simulink model "grid_afe_n"  (R2026a)
settings: Solver=ode23tb  StopTime=simlength  FixedStep=tc  MaxStep=glb_time.tc
values from neighbouring files (symbols this model uses):
  afe_ctrl = ctrl_afe_setup(glb_time.ts_afe, grid_emu.omega_grid_nom)    [init_model.m]
  afe_pwm_phase_shift_mod1 = 0    [init_model.m]
  afe_pwm_phase_shift_mod2 = 0    [init_model.m]
  afe_pwm_phase_shift_mod3 = 0    [init_model.m]
  afe_pwm_phase_shift_mod4 = 0    [init_model.m]
  filters = setup_global_filters(glb_time.ts_afe, glb_time.ts_inv, glb_time.ts_dab, glb_time.tc)    [init_model.m]
  frt_data = frt_settings(test_index, test_subindex, asymmetric_error_type,      enable_frt_1, enable_frt_2, start_time_LVRT, deepPOSxi, deepPOSeta, deepNEGxi, deepNEGeta)    [init_model.m]
  glb_time = timing_setup(fpwm_afe, trgo_afe, fpwm_inv, trgo_inv, fpwm_single_phase_inv, trgo_single_phase_inv, fpwm_dab, trgo_dab,      fpwm_psfbc, trgo_psfbc, fpwm_isop_rail, trgo_isop_rail, fpwm_cllc, trgo_cllc, t_measure, tc_factor, tc_decimation, delay_pwm, dead_time_afe,      dead_time_inv, dead_time_single_phase_inv, dead_time_dab, dead_time_psfbc, dead_time_isop_rail, dead_time_cllc)    [init_model.m]
  grid_emu = grid_three_phase_emulator('Dyn11', delta_star, grid_nominal_power, application_voltage, us1, us2, fgrid,                  eq_grid_inductance, eq_grid_resistance, eta, ucc, i1m, p_iron, n1, n2, core_area, core_length, mur,                  up_xi_pu_ref, up_eta_pu_ref, un_xi_pu_ref, un_eta_pu_ref)    [init_model.m]
  i_react_pos_ref_2 = -ixi_ref_mod1*tan(acos(0.95))    [init_model.m]
  i_react_pos_ref_3 = ixi_ref_mod1*tan(acos(0.95))    [init_model.m]
  ixi_ref_mod1 = -0.85    [init_model.m]
  ixi_ref_mod2 = -0.85    [init_model.m]
  ixi_ref_mod3 = -0.85    [init_model.m]
  ixi_ref_mod4 = -0.85    [init_model.m]
  ki_align = 18    [init_model.m]
  kp_align = 0.25    [init_model.m]
  lim_down_align = -0.05    [init_model.m]
  lim_up_align = 0.05    [init_model.m]
  mavarage_filter_frequency_base_order = 2    [init_model.m]
  time_gain_afe_module_1 = 1.0002    [init_model.m]
  time_gain_afe_module_2 = 1.0015    [init_model.m]
  time_gain_afe_module_3 = 0.9988    [init_model.m]
  time_gain_afe_module_4 = 1.0020    (= 1.002)    [init_model.m]
  time_i_react_pos_ref_1 = start_time_LVRT + error_length + 0.335    [init_model.m]
  time_i_react_pos_ref_2 = time_i_react_pos_ref_1 + 0.5    (= 0.5)    [init_model.m]
  u_cm_comp_mod1 = 0    [init_model.m]
  u_cm_comp_mod2 = -1    [init_model.m]
  u_cm_comp_mod3 = -1    [init_model.m]
  u_cm_comp_mod4 = -1    [init_model.m]
undefined symbols (not defined in the file or in its folder): hwdata, magnitude
libraries: fl_lib x113, nesl_utility x75, moving_average_filter x40, moving_average_filter_cc x32, sl_discontinuities x12, linear_double_integrator_observer_ccaller x8, discrete_time_low_pass_filter x4, threephase_inductor_lib x4, dclink_for_two_levels x4, three_phase_pwm_modulator x4, three_phase_inverter_ideal_switch_based_model x4, three_phase_inverter_igbt_advanced_thermal_model x4
(part 16 of 19)

== system grid_afe_n/afe_abc_mod4/AFE_control/afe_control/grid_voltage_phase_lock_loops/FHT-PLL/pll_stageA/filter_and_transformation ==
  ug_a : Inport
  ug_b : Inport  Port=2
  ug_c : Inport  Port=3
  Bus Creator : BusCreator  Inputs=2
  Bus Creator1 : BusCreator  Inputs=3
  Bus Creator2 : BusCreator  Inputs=2
  Bus Creator3 : BusCreator  Inputs=3
  Bus Creator4 : BusCreator  Inputs=3
  FHTalpha : Subsystem
  FHTbeta : Subsystem
  FHTdqPLL : Scope  NumInputPorts=2
      settings: ActiveDisplayYMinimum=-1.5258214459194912  ActiveDisplayYMaximum=1.5258228058860459  DataLoggingVariableName=ScopeData12
  Gain : Gain  Gain=-1/2
  Gain1 : Gain  Gain=-1/2
  Sum : Sum  Inputs=|++
  Sum1 : Sum  Inputs=-+|
  To Workspace1 : ToWorkspace  VariableName=ugd_alpha_sim  SampleTime=-1
      settings: MaxDataPoints=glb_time.Ns_afe
  To Workspace2 : ToWorkspace  VariableName=ugd_beta_sim  SampleTime=-1
      settings: MaxDataPoints=glb_time.Ns_afe
  To Workspace3 : ToWorkspace  VariableName=u_fht_alpha_sim  SampleTime=-1
      settings: MaxDataPoints=glb_time.Ns_afe
  To Workspace4 : ToWorkspace  VariableName=v_fht_alpha_sim  SampleTime=-1
      settings: MaxDataPoints=glb_time.Ns_afe
  To Workspace5 : ToWorkspace  VariableName=u_fhtsr_alpha_sim  SampleTime=-1
      settings: MaxDataPoints=glb_time.Ns_afe
  To Workspace6 : ToWorkspace  VariableName=u_fhtsr_beta_sim  SampleTime=-1
      settings: MaxDataPoints=glb_time.Ns_afe
  To Workspace7 : ToWorkspace  VariableName=u_fht_beta_sim  SampleTime=-1
      settings: MaxDataPoints=glb_time.Ns_afe
  To Workspace8 : ToWorkspace  VariableName=v_fht_beta_sim  SampleTime=-1
      settings: MaxDataPoints=glb_time.Ns_afe
  To Workspace9 : ToWorkspace  VariableName=ugd_abc_grid_sim  SampleTime=-1
      settings: MaxDataPoints=glb_time.Ns_afe
  abc2alphabeta : MATLAB Function  TreatAsAtomicUnit=on
  grid_voltages : Scope  NumInputPorts=3
      settings: ActiveDisplayYMinimum=-1.3618303835391998  ActiveDisplayYMaximum=1.3331545889377594  DataLoggingVariableName=ScopeData13
  ug_alpha : Outport  VectorParamsAs1DForOutWhenUnconnected=off
  ug_beta : Outport  Port=2  VectorParamsAs1DForOutWhenUnconnected=off
  wires:
  Bus Creator3/1 -> To Workspace9/1
  Bus Creator2/1 -> Bus Creator1/2  "FHTbeta"
  Bus Creator/1 -> Bus Creator4/2  "FHTalpha"
  Bus Creator4/1 -> FHTdqPLL/1
  Bus Creator1/1 -> FHTdqPLL/2
  FHTalpha/2(uq_hat) -> Bus Creator/2, To Workspace4/1, Sum1/1  "v_fht_alpha"
  FHTbeta/2(uq_hat) -> Bus Creator2/2, To Workspace8/1, Sum/2  "v_fht_beta"
  Gain/1 -> ug_alpha/1, To Workspace5/1, Bus Creator4/3  "u_fhtsr_alpha"
  Gain1/1 -> ug_beta/1, To Workspace6/1, Bus Creator1/3  "u_fhtsr_beta"
  Sum1/1 -> Gain1/1
  FHTbeta/1(ud_hat) -> Bus Creator2/1, To Workspace7/1, Sum1/2  "u_fht_beta"
  Sum/1 -> Gain/1
  FHTalpha/1(ud_hat) -> Sum/1, Bus Creator/1, To Workspace3/1  "u_fht_alpha"
  abc2alphabeta/2(beta) -> Bus Creator1/1, To Workspace2/1, FHTbeta/1(u)  "u_grid_beta"
  abc2alphabeta/1(alpha) -> Bus Creator4/1, FHTalpha/1(u), To Workspace1/1  "u_grid_alpha"
  ug_a/1 -> abc2alphabeta/1(a), grid_voltages/1, Bus Creator3/1  "ugd_a"
  ug_c/1 -> abc2alphabeta/3(c), grid_voltages/3, Bus Creator3/3  "ugd_c"
  ug_b/1 -> abc2alphabeta/2(b), grid_voltages/2, Bus Creator3/2  "ugd_b"

== system grid_afe_n/afe_abc_mod4/AFE_control/afe_control/grid_voltage_phase_lock_loops/FHT-PLL/pll_stageA/sequences ==
  u_grid_alpha : Inport
  u_grid_beta : Inport  Port=2
  phase_angle : Inport  Port=3
  alphabeta2xieta : MATLAB Function  TreatAsAtomicUnit=on
  u_grid_xi : Outport
  u_grid_eta : Outport  Port=2
  wires:
  phase_angle/1 -> alphabeta2xieta/3(gamma)  "phase_angle"
  u_grid_beta/1 -> alphabeta2xieta/2(beta)  "u_grid_beta"
  u_grid_alpha/1 -> alphabeta2xieta/1(alpha)  "u_grid_alpha"
  alphabeta2xieta/2(eta) -> u_grid_eta/1  "u_grid_eta"
  alphabeta2xieta/1(xi) -> u_grid_xi/1  "u_grid_xi"

== system grid_afe_n/afe_abc_mod4/AFE_control/afe_control/grid_voltage_phase_lock_loops/FHT-PLL/pll_stageB/double_integrator_observer ==
  theta : Inport
  Gain : Gain  Gain=afe_ctrl.di_obs.Ldso  Multiplication=Matrix(K*u)
  Gain1 : Gain  Gain=afe_ctrl.di_obs.Adso  Multiplication=Matrix(K*u)
  Gain2 : Gain  Gain=afe_ctrl.di_obs.Cso  Multiplication=Matrix(K*u)
  Selector : Selector  InputPortWidth=2  IndexOptions=Index vector (dialog)  Indices=2  OutputSizes=1
  Sum : Sum  Inputs=-+|
  Sum1 : Sum  Inputs=|++
  Unit Delay : UnitDelay  SampleTime=-1
  bounder1 : MATLAB Function  TreatAsAtomicUnit=on
  bounder2 : MATLAB Function  TreatAsAtomicUnit=on
  omega_hat : Outport
  wires:
  bounder2/1(y) -> Sum/1  "theta_hat_bounded"
  bounder1/1(y) -> Gain/1
  theta/1 -> Sum/2  "theta"
  Unit Delay/1 -> Gain2/1, Selector/1, Gain1/1
  Sum/1 -> bounder1/1(u)  "e"
  Sum1/1 -> Unit Delay/1
  Gain1/1 -> Sum1/2
  Gain2/1 -> bounder2/1(u)  "theta_hat"
  Selector/1 -> omega_hat/1
  Gain/1 -> Sum1/1

== system grid_afe_n/afe_abc_mod4/AFE_control/afe_control/grid_voltage_phase_lock_loops/FHT-PLL_simulink/pll_stageA/filter_and_transformation ==
  ug_a : Inport
  ug_b : Inport  Port=2
  ug_c : Inport  Port=3
  Bus Creator : BusCreator  Inputs=2
  Bus Creator1 : BusCreator  Inputs=3
  Bus Creator2 : BusCreator  Inputs=2
  Bus Creator4 : BusCreator  Inputs=3
  FHTalpha : Subsystem
  FHTbeta : Subsystem
  FHTdqPLL : Scope  NumInputPorts=2
      settings: ActiveDisplayYMinimum=-1.5258214459194912  ActiveDisplayYMaximum=1.5258228058860459  DataLoggingVariableName=ScopeData12
  Gain : Gain  Gain=-1/2
  Gain1 : Gain  Gain=-1/2
  Sum : Sum  Inputs=|++
  Sum1 : Sum  Inputs=-+|
  abc2alphabeta : MATLAB Function  TreatAsAtomicUnit=on
  grid_voltages : Scope  NumInputPorts=3
      settings: ActiveDisplayYMinimum=-1.3618303835391998  ActiveDisplayYMaximum=1.3331545889377594  DataLoggingVariableName=ScopeData13
  ug_alpha : Outport  VectorParamsAs1DForOutWhenUnconnected=off
  ug_beta : Outport  Port=2  VectorParamsAs1DForOutWhenUnconnected=off
  wires:
  Bus Creator2/1 -> Bus Creator1/2  "FHTbeta"
  Bus Creator/1 -> Bus Creator4/2  "FHTalpha"
  Bus Creator4/1 -> FHTdqPLL/1
  Bus Creator1/1 -> FHTdqPLL/2
  FHTalpha/2(ubeta) -> Bus Creator/2, Sum1/1  "v_fht_alpha"
  FHTbeta/2(ubeta) -> Bus Creator2/2, Sum/2  "v_fht_beta"
  Gain/1 -> ug_alpha/1, Bus Creator4/3  "u_fhtsr_alpha"
  Gain1/1 -> ug_beta/1, Bus Creator1/3  "u_fhtsr_beta"
  Sum1/1 -> Gain1/1
  FHTbeta/1(ualpha) -> Bus Creator2/1, Sum1/2  "u_fht_beta"
  Sum/1 -> Gain/1
  FHTalpha/1(ualpha) -> Sum/1, Bus Creator/1  "u_fht_alpha"
  abc2alphabeta/2(beta) -> FHTbeta/1(u), Bus Creator1/1  "u_grid_beta"
  abc2alphabeta/1(alpha) -> FHTalpha/1(u), Bus Creator4/1  "u_grid_alpha"
  ug_a/1 -> abc2alphabeta/1(a), grid_voltages/1  "ugd_a"
  ug_c/1 -> abc2alphabeta/3(c), grid_voltages/3  "ugd_c"
  ug_b/1 -> abc2alphabeta/2(b), grid_voltages/2  "ugd_b"

== system grid_afe_n/afe_abc_mod4/AFE_control/afe_control/grid_voltage_phase_lock_loops/FHT-PLL_simulink/pll_stageA/sequences ==
  u_grid_alpha : Inport
  u_grid_beta : Inport  Port=2
  phase_angle : Inport  Port=3
  alphabeta2xieta : MATLAB Function  TreatAsAtomicUnit=on
  u_grid_xi : Outport
  u_grid_eta : Outport  Port=2
  wires:
  phase_angle/1 -> alphabeta2xieta/3(gamma)  "phase_angle"
  u_grid_beta/1 -> alphabeta2xieta/2(beta)  "u_grid_beta"
  u_grid_alpha/1 -> alphabeta2xieta/1(alpha)  "u_grid_alpha"
  alphabeta2xieta/2(eta) -> u_grid_eta/1  "u_grid_eta"
  alphabeta2xieta/1(xi) -> u_grid_xi/1  "u_grid_xi"

== system grid_afe_n/afe_abc_mod4/AFE_control/afe_control/grid_voltage_phase_lock_loops/FHT-PLL_simulink/pll_stageB/double_integrator_observer ==
  theta : Inport
  Gain : Gain  Gain=afe_ctrl.di_obs.Ldso  Multiplication=Matrix(K*u)
  Gain1 : Gain  Gain=afe_ctrl.di_obs.Adso  Multiplication=Matrix(K*u)
  Gain2 : Gain  Gain=afe_ctrl.di_obs.Cso  Multiplication=Matrix(K*u)
  Selector : Selector  InputPortWidth=2  IndexOptions=Index vector (dialog)  Indices=2  OutputSizes=1
  Sum : Sum  Inputs=-+|
  Sum1 : Sum  Inputs=|++
  Unit Delay : UnitDelay  SampleTime=-1
  bounder1 : MATLAB Function  TreatAsAtomicUnit=on
  bounder2 : MATLAB Function  TreatAsAtomicUnit=on
  omega_hat : Outport
  wires:
  bounder2/1(y) -> Sum/1  "theta_hat_bounded"
  bounder1/1(y) -> Gain/1
  theta/1 -> Sum/2  "theta"
  Unit Delay/1 -> Gain2/1, Selector/1, Gain1/1
  Sum/1 -> bounder1/1(u)  "e"
  Sum1/1 -> Unit Delay/1
  Gain1/1 -> Sum1/2
  Gain2/1 -> bounder2/1(u)  "theta_hat"
  Selector/1 -> omega_hat/1
  Gain/1 -> Sum1/1

== system grid_afe_n/afe_abc_mod4/AFE_control/afe_control/grid_voltage_phase_lock_loops/dq_pll/pll_stageA/mormalization_and_transformation ==
  ug_a : Inport
  ug_b : Inport  Port=2
  ug_c : Inport  Port=3
  abc2alphabeta : MATLAB Function  TreatAsAtomicUnit=on
  ug_alpha : Outport  VectorParamsAs1DForOutWhenUnconnected=off
  ug_beta : Outport  Port=2  VectorParamsAs1DForOutWhenUnconnected=off
  wires:
  ug_c/1 -> abc2alphabeta/3(c)
  ug_b/1 -> abc2alphabeta/2(b)
  ug_a/1 -> abc2alphabeta/1(a)
  abc2alphabeta/1(alpha) -> ug_alpha/1  "u_grid_alpha"
  abc2alphabeta/2(beta) -> ug_beta/1  "u_grid_beta"

== system grid_afe_n/afe_abc_mod4/AFE_control/afe_control/grid_voltage_phase_lock_loops/dq_pll/pll_stageA/sequences ==
  u_grid_alpha : Inport
  u_grid_beta : Inport  Port=2
  gamma_grid : Inport  Port=3
  alphabeta2xieta : Subsystem
  u_grid_pos_xi : Outport
  u_grid_pos_eta : Outport  Port=2
  wires:
  gamma_grid/1 -> alphabeta2xieta/3(gamma)  "phase_grid"
  u_grid_beta/1 -> alphabeta2xieta/2(beta)  "u_grid_beta"
  u_grid_alpha/1 -> alphabeta2xieta/1(alpha)  "u_grid_alpha"
  alphabeta2xieta/2(eta) -> u_grid_pos_eta/1  "u_grid_pos_eta"
  alphabeta2xieta/1(xi) -> u_grid_pos_xi/1  "u_grid_pos_xi"

== system grid_afe_n/afe_abc_mod4/AFE_control/afe_control/grid_voltage_phase_lock_loops/dq_pll/pll_stageB/double_integrator_observer ==
  phase : Inport
  Gain : Gain  Gain=afe_ctrl.di_obs.Ldso  Multiplication=Matrix(K*u)
  Gain1 : Gain  Gain=afe_ctrl.di_obs.Adso  Multiplication=Matrix(K*u)
  Gain2 : Gain  Gain=afe_ctrl.di_obs.Cso  Multiplication=Matrix(K*u)
  Selector : Selector  InputPortWidth=2  IndexOptions=Index vector (dialog)  Indices=2  OutputSizes=1
  Sum : Sum  Inputs=-+|
  Sum1 : Sum  Inputs=|++
  Unit Delay : UnitDelay  SampleTime=-1
  bounder1 : MATLAB Function  TreatAsAtomicUnit=on
  bounder2 : MATLAB Function  TreatAsAtomicUnit=on
  omega_hat : Outport
  wires:
  bounder2/1(y) -> Sum/1  "theta_hat_bounded"
  bounder1/1(y) -> Gain/1  "e_bounded"
  phase/1 -> Sum/2  "phase"
  Unit Delay/1 -> Gain2/1, Selector/1, Gain1/1
  Sum/1 -> bounder1/1(u)  "e"
  Sum1/1 -> Unit Delay/1
  Gain1/1 -> Sum1/2
  Gain2/1 -> bounder2/1(u)  "theta_hat"
  Selector/1 -> omega_hat/1
  Gain/1 -> Sum1/1

== system grid_afe_n/afe_abc_mod4/AFE_control/afe_control/grid_voltage_phase_lock_loops/dq_pll/pll_stageB/scheduled-p-gain ==
  In1 : Inport
  Switch : Switch  Criteria=u2 > Threshold  Threshold=0.5  SaturateOnIntegerOverflow=off  InputSameDT=off
  kp1 : Gain  Gain=afe_ctrl.pll_p  SaturateOnIntegerOverflow=on  OutDataTypeStr=Inherit: Same as input  ParamDataTypeStr=Inherit: Same as input
  kp3 : Gain  Gain=afe_ctrl.pll_p_frt  SaturateOnIntegerOverflow=on  OutDataTypeStr=Inherit: Same as input  ParamDataTypeStr=Inherit: Same as input
  Out2 : Outport
  wires:
  Switch/1 -> Out2/1
  In1/1 -> kp3/1, kp1/1
  [frt_active] -> Switch/2
  kp1/1 -> Switch/3
  kp3/1 -> Switch/1

== system grid_afe_n/afe_abc_mod1/AFE_control/afe_control/current_ctrl/inner_current_ctrl/zero_current_ctrl/antiwind_up/anti_wind_up ==
  alpha : Inport
  beta : Inport  Port=2
  Saturation : Saturate  UpperLimit=10  LowerLimit=1
  Sqrt : Sqrt
  Square : Math  Operator=square
  Square1 : Math  Operator=square
  Sum : Sum  Inputs=|++
  scaling : Outport
  wires:
  alpha/1 -> Square/1
  Sum/1 -> Sqrt/1
  beta/1 -> Square1/1
  Square/1 -> Sum/1
  Square1/1 -> Sum/2
  Sqrt/1 -> Saturation/1
  Saturation/1 -> scaling/1

== system grid_afe_n/afe_abc_mod1/AFE_control/afe_control/grid_voltage_phase_lock_loops/FHT-PLL/pll_stageA/filter_and_transformation/FHTalpha ==
  u : Inport
  Bus Selector : BusSelector  OutputSignals=output_pu_hat,output_pu_hat_dot
  C Caller : CCaller  FunctionName=first_harmonic_tracker_process_simulink  PortSpecificationStruct="%)30     .    B \\   8    (     @         %    \"     D    !     0         %  0 \"0    $    _    07)G3F%M90  4&]R=$YA;64 4V-O<&4     26YD97@     5'EP90      4VEZ90      27-';&]B86P   X    P    !@    @    $          4    (     0    ,    !         !   P!O=70 #@   #     &    \"     0         !0    @    !     P    $         $  # &]U=  .    .     8    (    !          %    \"     $    &     0         0  ...(+4988 chars)"
  Constant : Constant  Value=glb_time.ts_afe
  Constant1 : Constant  Value=12
  Constant4 : Constant  Value=afe_ctrl.fht_grid.omega_fht
  Constant5 : Constant  Value=afe_ctrl.fht_grid.delta_fht
  Constant6 : Constant  Value=afe_ctrl.fht_grid.Ld_fht(1)
  Constant7 : Constant  Value=afe_ctrl.fht_grid.Ld_fht(2)
  Data Type Conversion{1..2,6..9} (6 alike) : DataTypeConversion  OutDataTypeStr=single  SaturateOnIntegerOverflow=off  RndMeth=Floor
  Data Type Conversion10 : DataTypeConversion  OutDataTypeStr=double  SaturateOnIntegerOverflow=off  RndMeth=Floor
  Data Type Conversion3 : DataTypeConversion  OutDataTypeStr=uint8  SaturateOnIntegerOverflow=off  RndMeth=Floor
  Data Type Conversion4 : DataTypeConversion  OutDataTypeStr=double  SaturateOnIntegerOverflow=off  RndMeth=Floor
  Data Type Conversion5 : DataTypeConversion  OutDataTypeStr=uint8  SaturateOnIntegerOverflow=off  RndMeth=Floor
  Gain : Gain  Gain=1/afe_ctrl.fht_grid.omega_fht
  Step : Step  Time=0.0125  InitialValue=1  FinalValue=0
  ud_hat : Outport
  uq_hat : Outport  Port=2
  wires:
  Data Type Conversion9/1 -> C Caller/7
  Data Type Conversion8/1 -> C Caller/6
  Data Type Conversion7/1 -> C Caller/5
  Data Type Conversion6/1 -> C Caller/4
  Data Type Conversion5/1 -> C Caller/8
  Constant5/1 -> Data Type Conversion7/1
  Constant7/1 -> Data Type Conversion9/1
  Constant6/1 -> Data Type Conversion8/1
  Constant4/1 -> Data Type Conversion6/1
  Constant1/1 -> Data Type Conversion5/1
  Constant/1 -> Data Type Conversion1/1
  u/1 -> Data Type Conversion2/1
  Step/1 -> Data Type Conversion3/1
  Bus Selector/1 -> Data Type Conversion4/1  "<output_pu_hat>"
  C Caller/1 -> Bus Selector/1
  Data Type Conversion2/1 -> C Caller/2
  Data Type Conversion1/1 -> C Caller/3
  Data Type Conversion3/1 -> C Caller/1
  Data Type Conversion4/1 -> ud_hat/1
  Data Type Conversion10/1 -> Gain/1
  Bus Selector/2 -> Data Type Conversion10/1  "<output_pu_hat_dot>"
  Gain/1 -> uq_hat/1

== system grid_afe_n/afe_abc_mod1/AFE_control/afe_control/grid_voltage_phase_lock_loops/FHT-PLL/pll_stageA/filter_and_transformation/FHTbeta ==
  u : Inport
  Bus Selector : BusSelector  OutputSignals=output_pu_hat,output_pu_hat_dot
  C Caller : CCaller  FunctionName=first_harmonic_tracker_process_simulink  PortSpecificationStruct="%)30     .    B \\   8    (     @         %    \"     D    !     0         %  0 \"0    $    _    07)G3F%M90  4&]R=$YA;64 4V-O<&4     26YD97@     5'EP90      4VEZ90      27-';&]B86P   X    P    !@    @    $          4    (     0    ,    !         !   P!O=70 #@   #     &    \"     0         !0    @    !     P    $         $  # &]U=  .    .     8    (    !          %    \"     $    &     0         0  ...(+4988 chars)"
  Constant : Constant  Value=glb_time.ts_afe
  Constant1 : Constant  Value=14
  Constant4 : Constant  Value=afe_ctrl.fht_grid.omega_fht
  Constant5 : Constant  Value=afe_ctrl.fht_grid.delta_fht
  Constant6 : Constant  Value=afe_ctrl.fht_grid.Ld_fht(1)
  Constant7 : Constant  Value=afe_ctrl.fht_grid.Ld_fht(2)
  Data Type Conversion{1..2,6..9} (6 alike) : DataTypeConversion  OutDataTypeStr=single  SaturateOnIntegerOverflow=off  RndMeth=Floor
  Data Type Conversion10 : DataTypeConversion  OutDataTypeStr=double  SaturateOnIntegerOverflow=off  RndMeth=Floor
  Data Type Conversion3 : DataTypeConversion  OutDataTypeStr=uint8  SaturateOnIntegerOverflow=off  RndMeth=Floor
  Data Type Conversion4 : DataTypeConversion  OutDataTypeStr=double  SaturateOnIntegerOverflow=off  RndMeth=Floor
  Data Type Conversion5 : DataTypeConversion  OutDataTypeStr=uint8  SaturateOnIntegerOverflow=off  RndMeth=Floor
  Gain : Gain  Gain=1/afe_ctrl.fht_grid.omega_fht
  Step : Step  Time=0.0125  InitialValue=1  FinalValue=0
  ud_hat : Outport
  uq_hat : Outport  Port=2
  wires:
  Gain/1 -> uq_hat/1
  Bus Selector/2 -> Data Type Conversion10/1  "<output_pu_hat_dot>"
  Data Type Conversion10/1 -> Gain/1
  Data Type Conversion4/1 -> ud_hat/1
  Data Type Conversion3/1 -> C Caller/1
  Data Type Conversion1/1 -> C Caller/3
  Data Type Conversion2/1 -> C Caller/2
  C Caller/1 -> Bus Selector/1
  Bus Selector/1 -> Data Type Conversion4/1  "<output_pu_hat>"
  Step/1 -> Data Type Conversion3/1
  u/1 -> Data Type Conversion2/1
  Constant/1 -> Data Type Conversion1/1
  Constant1/1 -> Data Type Conversion5/1
  Constant4/1 -> Data Type Conversion6/1
  Constant6/1 -> Data Type Conversion8/1
  Constant7/1 -> Data Type Conversion9/1
  Constant5/1 -> Data Type Conversion7/1
  Data Type Conversion5/1 -> C Caller/8
  Data Type Conversion6/1 -> C Caller/4
  Data Type Conversion7/1 -> C Caller/5
  Data Type Conversion8/1 -> C Caller/6
  Data Type Conversion9/1 -> C Caller/7

== system grid_afe_n/afe_abc_mod1/AFE_control/afe_control/grid_voltage_phase_lock_loops/FHT-PLL_simulink/pll_stageA/filter_and_transformation/FHTalpha ==
  u : Inport
  Gain : Gain  Gain=afe_ctrl.fht_grid.Ld_fht  Multiplication=Matrix(K*u)
  Gain1 : Gain  Gain=afe_ctrl.fht_grid.Ad_fht  Multiplication=Matrix(K*u)
  Gain2 : Gain  Gain=afe_ctrl.fht_grid.Cfht  Multiplication=Matrix(K*u)
  Gain3 : Gain  Gain=1/afe_ctrl.fht_grid.omega_fht
  Selector : Selector  InputPortWidth=2  IndexOptions=Index vector (dialog)  Indices=1  OutputSizes=1
  Selector1 : Selector  InputPortWidth=2  IndexOptions=Index vector (dialog)  Indices=2  OutputSizes=1
  Sum : Sum  Inputs=-+|
  Sum1 : Sum  Inputs=|++
  Unit Delay : UnitDelay  SampleTime=-1
  ualpha : Outport
  ubeta : Outport  Port=2
  wires:
  u/1 -> Sum/2
  Unit Delay/1 -> Gain2/1, Selector1/1, Selector/1, Gain1/1
  Sum/1 -> Gain/1
  Sum1/1 -> Unit Delay/1
  Gain1/1 -> Sum1/2
  Gain2/1 -> Sum/1
  Selector/1 -> ualpha/1
  Gain/1 -> Sum1/1
  Selector1/1 -> Gain3/1
  Gain3/1 -> ubeta/1

== system grid_afe_n/afe_abc_mod1/AFE_control/afe_control/grid_voltage_phase_lock_loops/FHT-PLL_simulink/pll_stageA/filter_and_transformation/FHTbeta ==
  u : Inport
  Gain : Gain  Gain=afe_ctrl.fht_grid.Ld_fht  Multiplication=Matrix(K*u)
  Gain1 : Gain  Gain=afe_ctrl.fht_grid.Ad_fht  Multiplication=Matrix(K*u)
  Gain2 : Gain  Gain=afe_ctrl.fht_grid.Cfht  Multiplication=Matrix(K*u)
  Gain3 : Gain  Gain=1/afe_ctrl.fht_grid.omega_fht
  Selector : Selector  InputPortWidth=2  IndexOptions=Index vector (dialog)  Indices=1  OutputSizes=1
  Selector1 : Selector  InputPortWidth=2  IndexOptions=Index vector (dialog)  Indices=2  OutputSizes=1
  Sum : Sum  Inputs=-+|
  Sum1 : Sum  Inputs=|++
  Unit Delay : UnitDelay  SampleTime=-1
  ualpha : Outport
  ubeta : Outport  Port=2
  wires:
  Gain3/1 -> ubeta/1
  Selector1/1 -> Gain3/1
  Gain/1 -> Sum1/1
  Selector/1 -> ualpha/1
  Gain2/1 -> Sum/1
  Gain1/1 -> Sum1/2
  Sum1/1 -> Unit Delay/1
  Sum/1 -> Gain/1
  Unit Delay/1 -> Gain1/1, Selector/1, Selector1/1, Gain2/1
  u/1 -> Sum/2

== system grid_afe_n/afe_abc_mod1/AFE_control/afe_control/grid_voltage_phase_lock_loops/dq_pll/pll_stageA/sequences/alphabeta2xieta ==
  alpha : Inport
  beta : Inport  Port=2
  gamma : Inport  Port=3
  alphabeta2xieta_neg : MATLAB Function  TreatAsAtomicUnit=on
  alphabeta2xieta_pos : MATLAB Function  TreatAsAtomicUnit=on
  xi : Outport
  eta : Outport  Port=2
  Out3 : Outport  Port=3
  Out4 : Outport  Port=4
  wires:
  alpha/1 -> alphabeta2xieta_neg/1(alpha), alphabeta2xieta_pos/1(alpha)  "u_grid_alpha"
  beta/1 -> alphabeta2xieta_neg/2(beta), alphabeta2xieta_pos/2(beta)  "u_grid_beta"
  gamma/1 -> alphabeta2xieta_neg/3(gamma), alphabeta2xieta_pos/3(gamma)  "phase_grid"
  alphabeta2xieta_pos/1(xi) -> xi/1  "u_grid_pos_xi"
  alphabeta2xieta_pos/2(eta) -> eta/1  "u_grid_pos_eta"
  alphabeta2xieta_neg/1(xi) -> Out3/1  "u_grid_neg_xi"
  alphabeta2xieta_neg/2(eta) -> Out4/1  "u_grid_neg_eta"

== system grid_afe_n/afe_abc_mod2/AFE_control/afe_control/current_ctrl/inner_current_ctrl/zero_current_ctrl/antiwind_up/anti_wind_up ==
  alpha : Inport
  beta : Inport  Port=2
  Saturation : Saturate  UpperLimit=10  LowerLimit=1
  Sqrt : Sqrt
  Square : Math  Operator=square
  Square1 : Math  Operator=square
  Sum : Sum  Inputs=|++
  scaling : Outport
  wires:
  Saturation/1 -> scaling/1
  Sqrt/1 -> Saturation/1
  Square1/1 -> Sum/2
  Square/1 -> Sum/1
  beta/1 -> Square1/1
  Sum/1 -> Sqrt/1
  alpha/1 -> Square/1

== system grid_afe_n/afe_abc_mod2/AFE_control/afe_control/grid_voltage_phase_lock_loops/FHT-PLL/pll_stageA/filter_and_transformation/FHTalpha ==
  u : Inport
  Bus Selector : BusSelector  OutputSignals=output_pu_hat,output_pu_hat_dot
  C Caller : CCaller  FunctionName=first_harmonic_tracker_process_simulink  PortSpecificationStruct="%)30     .    B \\   8    (     @         %    \"     D    !     0         %  0 \"0    $    _    07)G3F%M90  4&]R=$YA;64 4V-O<&4     26YD97@     5'EP90      4VEZ90      27-';&]B86P   X    P    !@    @    $          4    (     0    ,    !         !   P!O=70 #@   #     &    \"     0         !0    @    !     P    $         $  # &]U=  .    .     8    (    !          %    \"     $    &     0         0  ...(+4988 chars)"
  Constant : Constant  Value=glb_time.ts_afe
  Constant1 : Constant  Value=12
  Constant4 : Constant  Value=afe_ctrl.fht_grid.omega_fht
  Constant5 : Constant  Value=afe_ctrl.fht_grid.delta_fht
  Constant6 : Constant  Value=afe_ctrl.fht_grid.Ld_fht(1)
  Constant7 : Constant  Value=afe_ctrl.fht_grid.Ld_fht(2)
  Data Type Conversion{1..2,6..9} (6 alike) : DataTypeConversion  OutDataTypeStr=single  SaturateOnIntegerOverflow=off  RndMeth=Floor
  Data Type Conversion10 : DataTypeConversion  OutDataTypeStr=double  SaturateOnIntegerOverflow=off  RndMeth=Floor
  Data Type Conversion3 : DataTypeConversion  OutDataTypeStr=uint8  SaturateOnIntegerOverflow=off  RndMeth=Floor
  Data Type Conversion4 : DataTypeConversion  OutDataTypeStr=double  SaturateOnIntegerOverflow=off  RndMeth=Floor
  Data Type Conversion5 : DataTypeConversion  OutDataTypeStr=uint8  SaturateOnIntegerOverflow=off  RndMeth=Floor
  Gain : Gain  Gain=1/afe_ctrl.fht_grid.omega_fht
  Step : Step  Time=0.0125  InitialValue=1  FinalValue=0
  ud_hat : Outport
  uq_hat : Outport  Port=2
  wires:
  Gain/1 -> uq_hat/1
  Bus Selector/2 -> Data Type Conversion10/1  "<output_pu_hat_dot>"
  Data Type Conversion10/1 -> Gain/1
  Data Type Conversion4/1 -> ud_hat/1
  Data Type Conversion3/1 -> C Caller/1
  Data Type Conversion1/1 -> C Caller/3
  Data Type Conversion2/1 -> C Caller/2
  C Caller/1 -> Bus Selector/1
  Bus Selector/1 -> Data Type Conversion4/1  "<output_pu_hat>"
  Step/1 -> Data Type Conversion3/1
  u/1 -> Data Type Conversion2/1
  Constant/1 -> Data Type Conversion1/1
  Constant1/1 -> Data Type Conversion5/1
  Constant4/1 -> Data Type Conversion6/1
  Constant6/1 -> Data Type Conversion8/1
  Constant7/1 -> Data Type Conversion9/1
  Constant5/1 -> Data Type Conversion7/1
  Data Type Conversion5/1 -> C Caller/8
  Data Type Conversion6/1 -> C Caller/4
  Data Type Conversion7/1 -> C Caller/5
  Data Type Conversion8/1 -> C Caller/6
  Data Type Conversion9/1 -> C Caller/7

== system grid_afe_n/afe_abc_mod2/AFE_control/afe_control/grid_voltage_phase_lock_loops/FHT-PLL/pll_stageA/filter_and_transformation/FHTbeta ==
  u : Inport
  Bus Selector : BusSelector  OutputSignals=output_pu_hat,output_pu_hat_dot
  C Caller : CCaller  FunctionName=first_harmonic_tracker_process_simulink  PortSpecificationStruct="%)30     .    B \\   8    (     @         %    \"     D    !     0         %  0 \"0    $    _    07)G3F%M90  4&]R=$YA;64 4V-O<&4     26YD97@     5'EP90      4VEZ90      27-';&]B86P   X    P    !@    @    $          4    (     0    ,    !         !   P!O=70 #@   #     &    \"     0         !0    @    !     P    $         $  # &]U=  .    .     8    (    !          %    \"     $    &     0         0  ...(+4988 chars)"
  Constant : Constant  Value=glb_time.ts_afe
  Constant1 : Constant  Value=14
  Constant4 : Constant  Value=afe_ctrl.fht_grid.omega_fht
  Constant5 : Constant  Value=afe_ctrl.fht_grid.delta_fht
  Constant6 : Constant  Value=afe_ctrl.fht_grid.Ld_fht(1)
  Constant7 : Constant  Value=afe_ctrl.fht_grid.Ld_fht(2)
  Data Type Conversion{1..2,6..9} (6 alike) : DataTypeConversion  OutDataTypeStr=single  SaturateOnIntegerOverflow=off  RndMeth=Floor
  Data Type Conversion10 : DataTypeConversion  OutDataTypeStr=double  SaturateOnIntegerOverflow=off  RndMeth=Floor
  Data Type Conversion3 : DataTypeConversion  OutDataTypeStr=uint8  SaturateOnIntegerOverflow=off  RndMeth=Floor
  Data Type Conversion4 : DataTypeConversion  OutDataTypeStr=double  SaturateOnIntegerOverflow=off  RndMeth=Floor
  Data Type Conversion5 : DataTypeConversion  OutDataTypeStr=uint8  SaturateOnIntegerOverflow=off  RndMeth=Floor
  Gain : Gain  Gain=1/afe_ctrl.fht_grid.omega_fht
  Step : Step  Time=0.0125  InitialValue=1  FinalValue=0
  ud_hat : Outport
  uq_hat : Outport  Port=2
  wires:
  Data Type Conversion9/1 -> C Caller/7
  Data Type Conversion8/1 -> C Caller/6
  Data Type Conversion7/1 -> C Caller/5
  Data Type Conversion6/1 -> C Caller/4
  Data Type Conversion5/1 -> C Caller/8
  Constant5/1 -> Data Type Conversion7/1
  Constant7/1 -> Data Type Conversion9/1
  Constant6/1 -> Data Type Conversion8/1
  Constant4/1 -> Data Type Conversion6/1
  Constant1/1 -> Data Type Conversion5/1
  Constant/1 -> Data Type Conversion1/1
  u/1 -> Data Type Conversion2/1
  Step/1 -> Data Type Conversion3/1
  Bus Selector/1 -> Data Type Conversion4/1  "<output_pu_hat>"
  C Caller/1 -> Bus Selector/1
  Data Type Conversion2/1 -> C Caller/2
  Data Type Conversion1/1 -> C Caller/3
  Data Type Conversion3/1 -> C Caller/1
  Data Type Conversion4/1 -> ud_hat/1
  Data Type Conversion10/1 -> Gain/1
  Bus Selector/2 -> Data Type Conversion10/1  "<output_pu_hat_dot>"
  Gain/1 -> uq_hat/1
